simulink model "Maneuver"  (R2023b)
settings: Solver=ode4  StartTime=0.0  StopTime=30  FixedStep=dt  RelTol=1e-3
InitFcn:
  | SimulationInitialization
StopFcn:
  | SimulationEnd
values from neighbouring files (symbols this model uses):
  C = GeneticOpt.C    [SimulationCostFunction.m]
  c = Sw/b    (= 0.841696750903)    [SimulationControlConfig16P.m]    (also in SimulationControlConfig16P_LEGACY.m; SimulationControlConfigTAILLESS.m = 0.354008438819; SimulationControlConfigUTAIL.m = 0.354008438819)
  CL_Limit = CL_Max    (= 0.54)    [SimulationControlConfig16P.m]    (also in SimulationControlConfig16P_LEGACY.m; SimulationControlConfigTAILLESS.m; SimulationControlConfigUTAIL.m = 0.53)
  CL_Max_Nom = 0.465    [SimulationControlConfig16P.m]    (also in SimulationControlConfig16P_LEGACY.m; SimulationControlConfigTAILLESS.m = 0.39; SimulationControlConfigUTAIL.m)
  CL_Min = 0    [SimulationControlConfig16P.m]    (also in SimulationControlConfig16P_LEGACY.m; SimulationControlConfigTAILLESS.m; SimulationControlConfigUTAIL.m)
  dCl_per_dFlap = 0.005581818    [SimulationControlConfig16P.m]    (also in SimulationControlConfig16P_LEGACY.m = 0; SimulationControlConfigTAILLESS.m = 0; SimulationControlConfigUTAIL.m = 0)
  dt = DLLSim.dt    [SimulationTimeStep.m]    (also in SimulationTrim.m = 0.02)
  ElevatorDeflectionRate = 15    [SimulationControlConfig16P.m]    (also in SimulationControlConfig16P_LEGACY.m = 12; SimulationControlConfigTAILLESS.m = 10; SimulationControlConfigUTAIL.m = 12)
  ElevatorMax = 25    [SimulationControlConfig16P.m]    (also in SimulationControlConfig16P_LEGACY.m; SimulationControlConfigTAILLESS.m; SimulationControlConfigUTAIL.m)
  ElevatorPower = -0.002209    [SimulationControlConfig16P.m]    (also in SimulationControlConfig16P_LEGACY.m; SimulationControlConfigTAILLESS.m = -0.002956; SimulationControlConfigUTAIL.m = -0.00205983)
  ElevatorTrim = -3.5    [SimulationControlConfig16P.m]    (also in SimulationControlConfig16P_LEGACY.m; SimulationControlConfigTAILLESS.m = -6; SimulationControlConfigUTAIL.m = -8)
  Fp_Elevator = 0.55*2*pi*PitchRateLpfCutoff*dt    [SimulationControlConfig16P.m]    (also in SimulationControlConfig16P_LEGACY.m; SimulationControlConfigTAILLESS.m; SimulationControlConfigUTAIL.m)
  Fp_Pitch_2 = 0.55*2*pi*PitchBandwidth*dt    [SimulationControlConfig16P.m]    (also in SimulationControlConfig16P_LEGACY.m; SimulationControlConfigTAILLESS.m; SimulationControlConfigUTAIL.m)
  LaunchRollingElevator = -1.5    [SimulationControlConfig16P.m]    (also in SimulationControlConfig16P_LEGACY.m; SimulationControlConfigTAILLESS.m = 1; SimulationControlConfigUTAIL.m = 1)
  LiftSlope = 0.064285    [SimulationControlConfig16P.m]    (also in SimulationControlConfig16P_LEGACY.m; SimulationControlConfigTAILLESS.m = 0.058631; SimulationControlConfigUTAIL.m)
  LPFclestInit = 0    [SimulationControlPre.m]
  LPFvRate2PitchInit = 0.1    [SimulationControlPre.m]
  m = 13.1784    [InertiaEstimatorBWB.m]    (also in SimulationControlConfig16P.m = MassBWB; SimulationControlConfig16P_LEGACY.m = MassBWB; SimulationControlConfigTAILLESS.m = Weight / 2.2; SimulationControlConfigUTAIL.m = Weight / 2.2)
  nMax_User = 2.6    [SimulationControlConfig16P.m]    (also in SimulationControlConfig16P_LEGACY.m; SimulationControlConfigTAILLESS.m = 2.5; SimulationControlConfigUTAIL.m = 2.5)
  nMin_User = -1.3    [SimulationControlConfig16P.m]    (also in SimulationControlConfig16P_LEGACY.m; SimulationControlConfigTAILLESS.m = -1; SimulationControlConfigUTAIL.m = -1)
  Pitch2ElevatorIntegratorInit = -4    [SimulationControlPre.m]
  PitchDamping = -1.2608    [SimulationControlConfig16P.m]    (also in SimulationControlConfig16P_LEGACY.m; SimulationControlConfigTAILLESS.m = -0.6814; SimulationControlConfigUTAIL.m)
  PitchDampingTrust = 0.3    [SimulationControlConfig16P.m]    (also in SimulationControlConfig16P_LEGACY.m = 0.2; SimulationControlConfigTAILLESS.m = 0; SimulationControlConfigUTAIL.m = 0)
  PitchMaxAccel = 1.0    (= 1)    [SimulationControlConfig16P.m]    (also in SimulationControlConfig16P_LEGACY.m = 1.2; SimulationControlConfigTAILLESS.m; SimulationControlConfigUTAIL.m = 1.1)
  PitchRateLpfCutoff = 3    [SimulationControlConfig16P.m]    (also in SimulationControlConfig16P_LEGACY.m; SimulationControlConfigTAILLESS.m; SimulationControlConfigUTAIL.m = 5)
  PitchRateMax_User = PitchRateMax_User/180*pi    (= 0.523598775598)    [SimulationControlConfig16P.m]    (also in SimulationControlConfig16P_LEGACY.m; SimulationControlConfigTAILLESS.m; SimulationControlConfigUTAIL.m)
  PitchStiffness = -0.0041    [SimulationControlConfig16P.m]    (also in SimulationControlConfig16P_LEGACY.m; SimulationControlConfigTAILLESS.m = -0.00225; SimulationControlConfigUTAIL.m = -0.00194915)
  Q = GeneticOpt.Q    [SimulationCostFunction.m]
  R = GeneticOpt.R    [SimulationCostFunction.m]
  RateLimitPitchRateAccel = 0    [SimulationControlPre.m]
  RollingElevator = 5    [SimulationControlConfig16P.m]    (also in SimulationControlConfig16P_LEGACY.m; SimulationControlConfigTAILLESS.m = 6.5; SimulationControlConfigUTAIL.m = 7)
  RotationElevator = -6.5    [SimulationControlConfig16P.m]    (also in SimulationControlConfig16P_LEGACY.m; SimulationControlConfigTAILLESS.m = -4.25; SimulationControlConfigUTAIL.m = -5.7)
  RotationRate = (RotationElevator - LaunchRollingElevator)/RotationTime    (= -1)    [SimulationControlConfig16P.m]    (also in SimulationControlConfig16P_LEGACY.m; SimulationControlConfigTAILLESS.m = -1.5; SimulationControlConfigUTAIL.m = -1.86111111111)
  Sw = 4.663    [SimulationControlConfig16P.m]    (also in SimulationControlConfig16P_LEGACY.m; SimulationControlConfigTAILLESS.m = 0.839; SimulationControlConfigUTAIL.m = 0.839)
  taxiTrackOffset = testPlans(testIndx).rolloutTrackOffset    [SimulationControlConfig16P.m]    (also in SimulationControlConfig16P_LEGACY.m; SimulationControlConfigTAILLESS.m; SimulationControlConfigUTAIL.m)
  YInertia = 134.120    (= 134.12)    [SimulationControlConfig16P.m]    (also in SimulationControlConfig16P_LEGACY.m; SimulationControlConfigTAILLESS.m = IYY / 3417.17; SimulationControlConfigUTAIL.m = IYY / 3417.17)
undefined symbols (not defined in the file or in its folder): DiscIntNeverNeededParam, gain_resolution, K_TS, KI_Pitch, KP_Pitch, PB, pilotTime, stepTime
libraries: simulink x22, Lib_Piccolo x18, simulink_extras x1
(part 2 of 2)

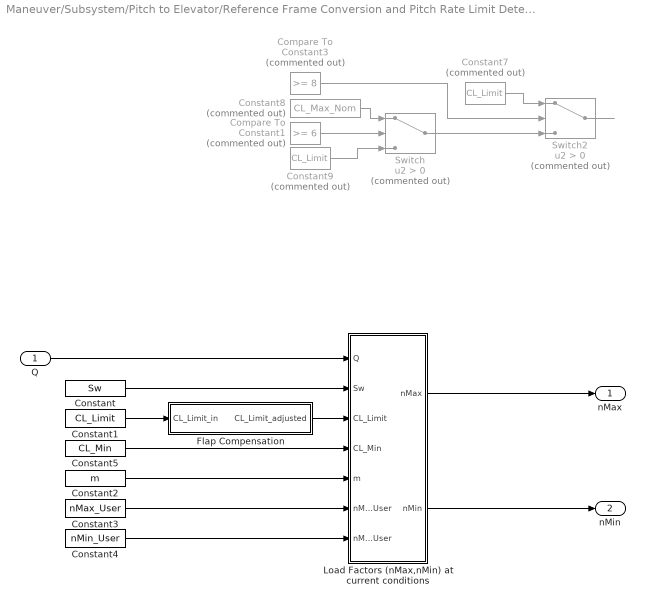
== system Maneuver/Subsystem/Pitch to Elevator/Reference Frame Conversion and Pitch Rate Limit Determination/AeroVsStruct_Limit ==
  Q : Inport
  Compare To Constant1 : simulink/Logic and Bit Operations/Compare To Constant  Commented=on  relop=>=  const=6  OutDataTypeStr=uint8
  Compare To Constant3 : simulink/Logic and Bit Operations/Compare To Constant  Commented=on  relop=>=  const=8  OutDataTypeStr=uint8
  Constant : Constant  Value=Sw
  Constant1 : Constant  Value=CL_Limit
  Constant2 : Constant  Value=m
  Constant3 : Constant  Value=nMax_User
  Constant4 : Constant  Value=nMin_User
  Constant5 : Constant  Value=CL_Min
  Constant7 : Constant  Commented=on  Value=CL_Limit
  Constant8 : Constant  Commented=on  Value=CL_Max_Nom
  Constant9 : Constant  Commented=on  Value=CL_Limit
  Flap Compensation : Subsystem
  "Load Factors (nMax,nMin) at current conditions " : MATLAB Function  TreatAsAtomicUnit=on
  Switch : Switch  Commented=on  Criteria=u2 > Threshold  SaturateOnIntegerOverflow=off  InputSameDT=off
  Switch2 : Switch  Commented=on  Criteria=u2 > Threshold  SaturateOnIntegerOverflow=off  InputSameDT=off
  nMax : Outport  VectorParamsAs1DForOutWhenUnconnected=off
  "nMin " : Outport  Port=2  VectorParamsAs1DForOutWhenUnconnected=off
  wires:
  Constant9/1 -> Switch/3
  Switch2/1 -> ?
  Switch/1 -> Switch2/3
  Compare To Constant1/1 -> Switch/2
  Constant7/1 -> Switch2/1
  Constant8/1 -> Switch/1
  Compare To Constant3/1 -> Switch2/2
  Q/1 -> "Load Factors (nMax,nMin) at current conditions "/1(Q)
  "Load Factors (nMax,nMin) at current conditions "/1(nMax) -> nMax/1
  Constant/1 -> "Load Factors (nMax,nMin) at current conditions "/2(Sw)
  Constant2/1 -> "Load Factors (nMax,nMin) at current conditions "/5(m)
  Constant3/1 -> "Load Factors (nMax,nMin) at current conditions "/6(nMax_User)
  Constant4/1 -> "Load Factors (nMax,nMin) at current conditions "/7(nMin_User)
  Constant5/1 -> "Load Factors (nMax,nMin) at current conditions "/4(CL_Min)
  "Load Factors (nMax,nMin) at current conditions "/2(nMin) -> "nMin "/1
  Constant1/1 -> Flap Compensation/1(CL_Limit_in)
  Flap Compensation/1(CL_Limit_adjusted) -> "Load Factors (nMax,nMin) at current conditions "/3(CL_Limit)

== system Maneuver/Subsystem/Pitch to Elevator/TASLimit/Latch ==
  D : Inport
  Enable/!Rst : Inport  Port=2
  AND : Logic  IconShape=distinctive  AllPortsSameDT=off  OutDataTypeStr=boolean
  Constant : Constant
  OR : Logic  Operator=OR  IconShape=distinctive  AllPortsSameDT=off  OutDataTypeStr=boolean
  Switch : Switch  Criteria=u2 > Threshold  Threshold=0.5  SaturateOnIntegerOverflow=off  InputSameDT=off
  Unit Delay : UnitDelay  SampleTime=-1  HasFrameUpgradeWarning=on
  Q_Latched : Outport  VectorParamsAs1DForOutWhenUnconnected=off
  wires:
  Unit Delay/1 -> OR/2
  Switch/1 -> Q_Latched/1, Unit Delay/1
  D/1 -> Switch/3, OR/1
  OR/1 -> AND/1
  AND/1 -> Switch/2
  Enable/!Rst/1 -> AND/2
  Constant/1 -> Switch/1

== system Maneuver/Subsystem/Pitch to Elevator/Reference Frame Conversion and Pitch Rate Limit Determination/AeroVsStruct_Limit/Flap Compensation ==
  CL_Limit_in : Inport
  Gain : Gain  Gain=dCl_per_dFlap
  Sum : Sum  Inputs=|++
  CL_Limit_adjusted : Outport  VectorParamsAs1DForOutWhenUnconnected=off
  wires:
  CL_Limit_in/1 -> Sum/1
  Sum/1 -> CL_Limit_adjusted/1
  Gain/1 -> Sum/2
  [flapCmd] -> Gain/1

== matlab function Maneuver/Subsystem/Pitch to Elevator/Reference Frame Conversion and Pitch Rate Limit Determination/AeroVsStruct_Limit/Load Factors (nMax,nMin) at current conditions  ==
  data: Q input; nMax output; Sw input; CL_Limit input; CL_Min input; m input; nMax_User input; nMin_User input; nMin output
function [nMax, nMin] = fcn(Q, Sw, CL_Limit,CL_Min, m, nMax_User, nMin_User)

nAero_Max=Sw*Q*CL_Limit/(m*9.81);
nAero_Min=Sw*Q*CL_Min/(m*9.81);
nMax=min(nMax_User,nAero_Max);
nMin=max(nMin_User, nAero_Min);
end

== matlab function Maneuver/Subsystem/Pitch to Elevator/Reference Frame Conversion and Pitch Rate Limit Determination/MATLAB Function ==
  data: PitchCmd_Euler input; PitchCmd_Body output; Pitch_Euler input; Roll_Euler input; Pitch_Body output; Scalar output; PitchRateCmd_Body output; PitchRateLimit_Max output; PitchRateLimit_Min output; V input; nMax input; nMin input; PitchRateMax_User input; nPrime_Max output; nPrime_Min output
function [PitchCmd_Body,Pitch_Body, Scalar, PitchRateCmd_Body, PitchRateLimit_Max, PitchRateLimit_Min,nPrime_Max,nPrime_Min] = fcn(PitchCmd_Euler, Pitch_Euler, Roll_Euler,V,nMax,nMin,PitchRateMax_User)
g=9.81;
cPhi=cos(Roll_Euler); % input should be in radian
if (0<=cPhi)&&(cPhi<0.5)
    cPhi=0.5;
elseif (0>cPhi)&&(cPhi>-0.5)
    cPhi=-0.5;
end
Scalar=1/cPhi;
PitchCmd_Body=PitchCmd_Euler*Scalar;
Pitch_Body=Pitch_Euler*Scalar;
% PitchRateCmd_Body=abs(sin(Roll_Euler))*g/(cPhi*V); 
PitchRateCmd_Body=(sin(Roll_Euler))^2*g/(cPhi*V); 
%PitchRateCmd_Body=sin(Roll_Euler)^2*g/(cPhi^2*V); 
% error in the documentation
% Wrong in the documentation !
% nPrime_Max=nMax*(1-g)*cos(Roll_Euler)*cos(Pitch_Euler); 
% nPrime_Min=nMin*(1-g)*cos(Roll_Euler)*cos(Pitch_Euler);
nPrime_Max=(nMax-1)*cos(Roll_Euler)*cos(Pitch_Euler);
nPrime_Min=(nMin-1)*cos(Roll_Euler)*cos(Pitch_Euler);

PitchRateLimit_Max=min(PitchRateCmd_Body+PitchRateMax_User, g*nPrime_Max/V);
PitchRateLimit_Min=max(PitchRateCmd_Body-PitchRateMax_User, g*nPrime_Min/V);

% PitchRateLimit_Max=PitchRateMax_User;
% PitchRateLimit_Min=-PitchRateMax_User;
% PitchRateLimit_Max=PitchRateCmd_Body+PitchRateMax_User;
% PitchRateLimit_Min=PitchRateCmd_Body-PitchRateMax_User;
end
